simulink model "meteorprocess_model3"  (R2022b)
settings: Solver=VariableStepAuto  StartTime=0.0  StopTime=10  RelTol=1e-3
libraries: audiosources x1, dspsnks4 x1, dsparch4 x1
settings Model: Creator=bruce  LastModifiedBy=bruce

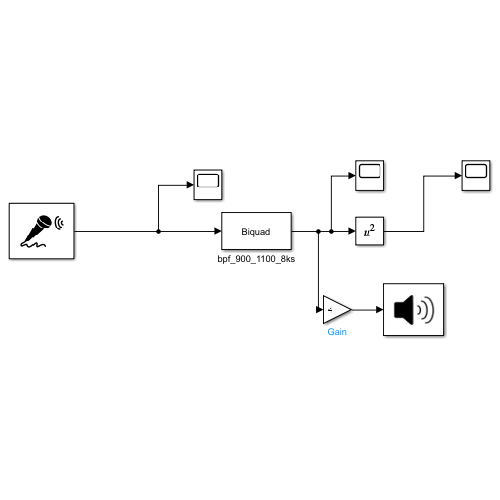
[thumbnail: Simulink's stored preview of the top-level diagram]
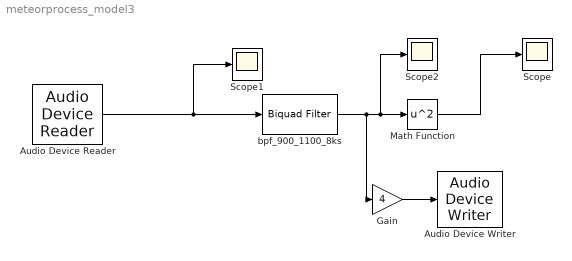
== system meteorprocess_model3 ==
  Audio Device Reader : audiosources/Audio Device Reader  Driver=DirectSound  Device=Microphone (Logitech USB Headset)  SampleRate=8000  NumChannels=1  SamplesPerFrame=1024  BitDepth=16-bit integer  NumBuffers=10  DefaultInputChannelMapping=on  InputChannelMapping=1:2  OutputNumOverrunSamples=off  OutputDataType=double  DriverIdx=1  DeviceWarnFlag=''
  Audio Device Writer : dspsnks4/Audio Device Writer  Driver=DirectSound  Device=Speakers (Logitech USB Headset)  InheritSampleRate=off  SampleRate=8000  BitDepth=16-bit integer  BufferSize=4096  NumBuffers=10  DefaultOutputChannelMapping=on  OutputChannelMapping=1:2  OutputNumUnderrunSamples=off  DriverIdx=1  DeviceWarnFlag=''
  Gain : Gain  Gain=4
  Math Function : Math  Operator=square
  Scope : Scope
  Scope1 : Scope
  Scope2 : Scope
  bpf_900_1100_8ks : dsparch4/Biquad Filter  Tag=BlockMethodSubSystem  FilterSource=Dialog parameters  CoeffSource=Specify via dialog  FilterObject=BQF  IIRFiltStruct=Direct form II  BiQuadCoeffs=[1 0 -1 1 -1.26776065363229673 0.937718928516803718;1 0 -1 1 -1.47280713132879892 0.945947631723422666;1 0 -1 1 -1.27886838367545685 0.860715192436244836;1 0 -1 1 -1.36391119365840674 0.868402670797701504]  ScaleValues=[0.0762110680568440224;0.0762110680568440224;0.0733382179883900753;0.0733382179883900753;1]  IC=0  ICnum=0  ICden=0  a0Flag=Warning  optimizeScaleValues=on  ScaleValueMode=Specify via input port (g)  InputProcessing=Columns as channels (frame based)  roundingMode=Floor  overflowMode=off  scaleValueFracLength=14  denProdOutputFracLength=30  denAccumFracLength=30  secondMemoryFracLength=15
  wires:
  bpf_900_1100_8ks/1 -> Gain/1, Scope2/1, Math Function/1
  Audio Device Reader/1 -> bpf_900_1100_8ks/1, Scope1/1
  Math Function/1 -> Scope/1
  Gain/1 -> Audio Device Writer/1
